simulink subsystem "AdmittanceExecution"  (R2025b)
settings: Solver=VariableStepAuto  StartTime=0.0  StopTime=10.0  RelTol=1e-3
undefined symbols (not defined in the file): controlRobot, lambda
settings Model: Creator=Compu  LastModifiedBy=Compu

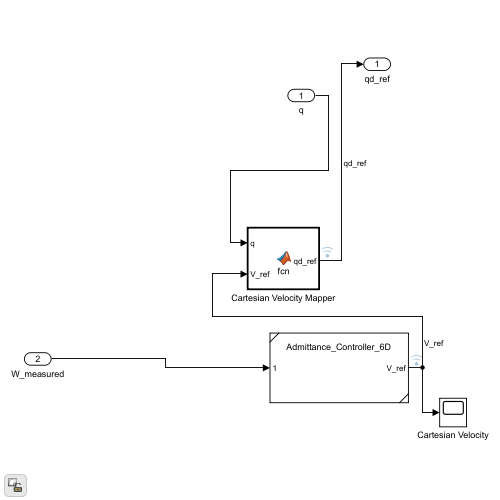
[thumbnail: Simulink's stored preview of the top-level diagram]
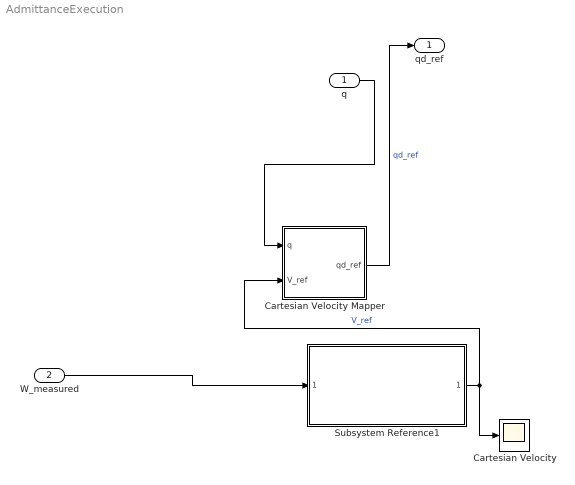
== system AdmittanceExecution ==
  q : Inport
  W_measured : Inport  Port=2
  Cartesian Velocity : Scope
      settings: ActiveDisplayYMinimum=-1  ActiveDisplayYMaximum=1
  Cartesian Velocity Mapper : MATLAB Function  TreatAsAtomicUnit=on
  Subsystem Reference1 : Subsystem  ReferencedSubsystem=Admittance_Controller_6D
  qd_ref : Outport
  wires:
  Subsystem Reference1/1 -> Cartesian Velocity/1, Cartesian Velocity Mapper/2(V_ref)  "V_ref"
  q/1 -> Cartesian Velocity Mapper/1(q)
  Cartesian Velocity Mapper/1(qd_ref) -> qd_ref/1  "qd_ref"
  W_measured/1 -> Subsystem Reference1/1

== matlab function AdmittanceExecution/Cartesian Velocity Mapper ==
  data: q input; V_ref input; controlRobot parameter; lambda parameter; qd_ref output double size=[6 1]
function qd_ref  = fcn(q, V_ref, controlRobot, lambda)

qd_ref = cartesianVelocityMapper( ...
    controlRobot, q, V_ref, lambda);

end
